simulink model "AC_DCj_iaocuo_full_TCM_THD_optimized_"  (R2024b)
settings: Solver=FixedStepDiscrete  StartTime=0.0  StopTime=0.2  FixedStep=1e-7  RelTol=1e-3
libraries: spsMosfetLib x6, spsSeriesRLCBranchLib x6, spsCurrentMeasurementLib x4, spsVoltageMeasurementLib x2, spsACVoltageSourceLib x1, slpidlib x1, dspstat3 x1, sps_lib x1, simulink x1
settings Model: Creator=YuJian  LastModifiedBy=YuJian
settings DataIOCC: ReturnWorkspaceOutputs=off

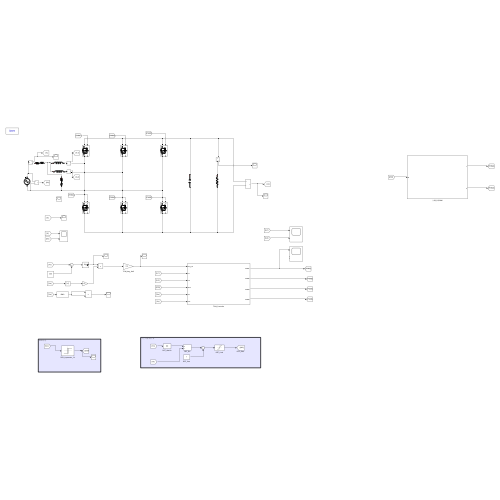
[thumbnail: Simulink's stored preview of the top-level diagram]
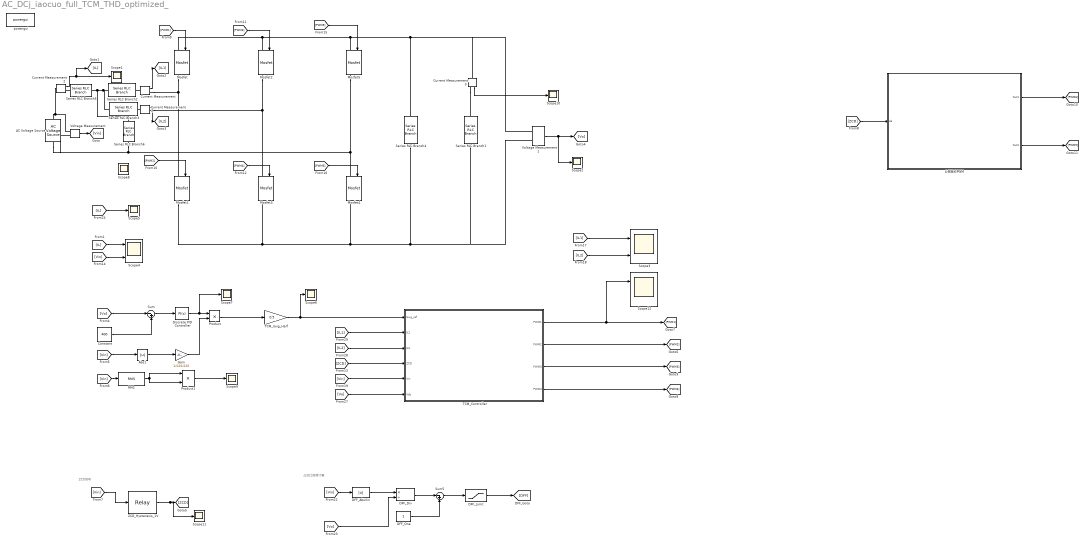
== system AC_DCj_iaocuo_full_TCM_THD_optimized_ ==
  note: 占空比前馈计算
  note: ZCD信号
  AC Voltage Source : spsACVoltageSourceLib/AC Voltage Source  Amplitude=311  Phase=0  Frequency=50  SampleTime=0  Measurements=None  BusType=swing  Pref=10e3  Qref=0  Qmin=-inf  Qmax=+inf
  Abs1 : Abs  SaturateOnIntegerOverflow=off
  Constant : Constant  Value=400
  Current Measurement{,1..3} (4 alike) : spsCurrentMeasurementLib/Current Measurement  PhasorSimulation=off  OutputType=Complex  PSBequivalent=0
  DFF_AbsVin : Abs  SaturateOnIntegerOverflow=off
  DFF_Div : Product  Inputs=*/
  DFF_Limit : Saturate  UpperLimit=1  LowerLimit=0
  DFF_One : Constant
  Discrete PID Controller : slpidlib/PID Controller  Controller=PI  Form=Parallel  TimeDomain=Discrete-time  UseExternalTs=off  SampleTime=-1  IntegratorMethod=Forward Euler  FilterMethod=Forward Euler  ControllerParametersSource=internal  P=4  I=230  UseKiTs=off  D=0  UseExternalDerivativeSource=off  N=100  UseFilter=on  TunerSelectOption=Transfer Function Based (PID Tuner App)  InitialConditionSource=internal  InitialConditionForIntegrator=5500  InitialConditionForFilter=0  DifferentiatorICPrevScaledInput=0  ExternalReset=none  TrackingMode=off  Kt=1  LimitOutput=on  SatLimitsSource=internal  UpperSaturationLimit=6500  LowerSaturationLimit=0  LinearizeAsGain=off  AntiWindupMode=clamping  Kb=1  LimitIntegrator=off  UpperIntegratorSaturationLimit=inf  LowerIntegratorSaturationLimit=-inf  POutMin=[]  POutMax=[]  IOutMin=[]  IOutMax=[]  DOutMin=[]  DOutMax=[]  NOutMin=[]  NOutMax=[]  SumOutMin=[]  SumOutMax=[]  SaturationOutMin=[]  SaturationOutMax=[]  PParamMin=[]  PParamMax=[]  IParamMin=[]  IParamMax=[]  DParamMin=[]  DParamMax=[]  NParamMin=[]  NParamMax=[]  KbParamMin=[]  KbParamMax=[]  KtParamMin=[]  KtParamMax=[]  KbOutMin=[]  KbOutMax=[]  KtOutMin=[]  KtOutMax=[]  IntegratorOutMin=[]  IntegratorOutMax=[]  FilterOutMin=[]  FilterOutMax=[]  SumI1OutMin=[]  SumI1OutMax=[]  SumI2OutMin=[]  SumI2OutMax=[]  SumI3OutMin=[]  SumI3OutMax=[]  SumI4OutMin=[]  SumI4OutMax=[]  SumDOutMin=[]  SumDOutMax=[]  DifferentiatorOutMin=[]  DifferentiatorOutMax=[]  FilterDiffOutCoefMin=[]  FilterDiffOutCoefMax=[]  ReciprocalOutMin=[]  ReciprocalOutMax=[]  SumDenOutMin=[]  SumDenOutMax=[]  SumNumOutMin=[]  SumNumOutMax=[]  DivideOutMin=[]  DivideOutMax=[]  UdiffTsProdOutMin=[]  UdiffTsProdOutMax=[]  NTsProdOutMin=[]  NTsProdOutMax=[]  UintegralTsProdOutMin=[]  UintegralTsProdOutMax=[]  UngainTsProdOutMin=[]  UngainTsProdOutMax=[]  ClampingZeroOutDataTypeStr=Inherit: Inherit via back propagation  ClampingZeroOutMin=[]  ClampingZeroOutMax=[]  FilterDenConstantOutDataTypeStr=Inherit: Inherit via back propagation  FilterDenConstantOutMin=[]  FilterDenConstantOutMax=[]  PCopyOutDataTypeStr=Inherit: Inherit via back propagation  PCopyOutMin=[]  PCopyOutMax=[]  NCopyOutDataTypeStr=Inherit: Inherit via back propagation  NCopyOutMin=[]  NCopyOutMax=[]  IntegratorContinuousStateAttributes=''  IntegratorStateMustResolveToSignalObject=off  IntegratorRTWStateStorageClass=Auto  FilterContinuousStateAttributes=''  FilterStateMustResolveToSignalObject=off  FilterRTWStateStorageClass=Auto  ParallelPVariant=InternalParameters  IdealPVariant=Disabled  IVariant=InternalParameters  DVariant=Disabled  IntegratorVariant=Discrete  SatVariant=Enabled  AWVariant=DiscClampingParallel  PCopyVariant=Disabled  TRVariant=Disabled  FdbkBlocksVariant=Forward  IdealPFdbkVariant=Disabled  SatFdbkVariant=Disabled  DerivativeFilterVariant=Disabled  NVariant=Disabled  NCopyVariant=Disabled_SignalSpec  FilterICVariant=Disabled  IntegratorICVariant=InternalICs  ExternalResetVariant=Disabled  TRSumVariant=Passthrough  SumFdbkVariant=Disabled  SumVariant=Sum_PI  TsampFilterVariant=InternalTs  TsampNgainVariant=Passthrough  TsampIntegralVariant=Disabled_SignalSpec  ExternalSaturationOutDataTypeStr=Inherit: Same as second input  DerivativeSourceVariant=Disabled  PreIntVariant=InternalPreInt
      settings: LibrarySourceBlock=simulink/Discrete/Discrete PID Controller
  Gain : Gain  Gain=1/220/220
  Mosfet{,1..5} (6 alike) : spsMosfetLib/Mosfet  Ron=0.1  Lon=0  Rd=0.01  Vfd=0  IC=0  Rs=1e5  Cs=inf  Measurements=on
  Product : Product
  Product1 : Product
  RMS : dspstat3/RMS  run=off  directionMode=Each column  dimension=1  InputProcessing=Columns as channels (frame based)  reset_popup=None
  Scope{1..2,5..11} (9 alike) : Scope
  Scope12 : Scope  NumInputPorts=2
  Scope3 : Scope  NumInputPorts=2
  Scope4 : Scope  NumInputPorts=2
  Series RLC Branch1 : spsSeriesRLCBranchLib/Series RLC Branch  LConnTagsString=__new0  RConnTagsString=__new0  BranchType=R  Resistance=29.0909  Inductance=1e-3  SetiL0=off  InitialCurrent=0  Capacitance=1e-6  Setx0=off  InitialVoltage=0  Measurements=None
  Series RLC Branch2 : spsSeriesRLCBranchLib/Series RLC Branch  LConnTagsString=__new0  RConnTagsString=__new0  BranchType=L  Resistance=1  Inductance=50e-6  SetiL0=off  InitialCurrent=0  Capacitance=1e-6  Setx0=off  InitialVoltage=0  Measurements=None
  Series RLC Branch3 : spsSeriesRLCBranchLib/Series RLC Branch  LConnTagsString=__new0  RConnTagsString=__new0  BranchType=L  Resistance=1  Inductance=50e-6  SetiL0=off  InitialCurrent=0  Capacitance=1e-6  Setx0=off  InitialVoltage=0  Measurements=None
  Series RLC Branch4 : spsSeriesRLCBranchLib/Series RLC Branch  LConnTagsString=__new0  RConnTagsString=__new0  BranchType=C  Resistance=1  Inductance=1e-3  SetiL0=off  InitialCurrent=0  Capacitance=2680e-6  Setx0=on  InitialVoltage=400  Measurements=None
  Series RLC Branch5 : spsSeriesRLCBranchLib/Series RLC Branch  LConnTagsString=__new0  RConnTagsString=__new0  BranchType=RL  Resistance=0.05  Inductance=30e-6  SetiL0=off  InitialCurrent=0  Capacitance=1e-6  Setx0=off  InitialVoltage=0  Measurements=None
  Series RLC Branch6 : spsSeriesRLCBranchLib/Series RLC Branch  LConnTagsString=__new0  RConnTagsString=__new0  BranchType=RC  Resistance=1  Inductance=30e-6  SetiL0=off  InitialCurrent=0  Capacitance=2.2e-6  Setx0=off  InitialVoltage=0  Measurements=None
  Sum : Sum  Inputs=|-+
  Sum5 : Sum  Inputs=|-+
  TCM_Controller : Subsystem
  TCM_Iavg_Half : Gain  Gain=0.5
  Voltage Measurement : spsVoltageMeasurementLib/Voltage Measurement  PhasorSimulation=off  OutputType=Complex  PSBequivalent=0
  Voltage Measurement1 : spsVoltageMeasurementLib/Voltage Measurement  PhasorSimulation=off  OutputType=Complex  PSBequivalent=0
  ZCD_Hysteresis_1V : Relay  OnSwitchValue=1  OffSwitchValue=-1  OutDataTypeStr=boolean
  powergui : sps_lib/powergui  Priority=1  SimulationMode=Discrete  SampleTime=1e-7  frequency=60  Iterations=50  frequencyindice=50  Pbase=100e6  ErrMax=1e-4  UnitsV=kV  UnitsW=MW  buscounter=0  FunctionMessages=off  echomessages=off  EnableUseOfTLC=off  CurrentSourceSwitches=off  DisableSnubberDevices=off  DisableRonSwitches=off  DisableVfSwitches=off  DisplayEquations=off  AutomaticDiscreteSolvers=off  SolverType=Tustin/Backward Euler (TBE)  Interpol=off  ExternalGateDelay=off  methode=off  Ts=100  x0status=blocks  SPID=on  SwTol=0  HookPort=off  NonlinearTolerance=1e-4  nMaxIteration=100  ContinueOnMaxIteration=off  RestoreLinks=warning  ResistiveCurrentMeasurement=off  Frange=[0:2:500]  Ylog=off  Xlog=on  ShowGrid=off  save=off  variable=ZData  structure=0  ZoomFFT=off  StartTime=0.0  cycles=1  DisplayStyle=1  fundamental=60  FreqAxis=off  MaxFrequency=1000  frequencyindicesteady=1  RmsSteady=1  display=off
  公频驱动PWM : Subsystem
  wires:
  Current Measurement2/1 -> Scope1/1, [IL]
  Current Measurement/1 -> [IL1]
  Current Measurement1/1 -> [IL2]
  Voltage Measurement1/1 -> Scope2/1, [Vo]
  Voltage Measurement/1 -> [Vin]
  Constant/1 -> Sum/2
  [Vo] -> Sum/1
  Sum/1 -> Discrete PID Controller/1
  Discrete PID Controller/1 -> Scope7/1, Product/1
  Gain/1 -> Product/2
  [Vin] -> RMS/1
  [PWM4] -> Mosfet3/1
  [PWM3] -> Mosfet2/1
  [PWM2] -> Mosfet1/1
  [PWM1] -> Mosfet/1
  [PWM5] -> Mosfet5/1
  [PWM6] -> Mosfet4/1
  [IL1] -> Scope3/1
  [IL2] -> Scope3/2
  Product1/1 -> Scope9/1
  Current Measurement3/1 -> Scope10/1
  [Vin] -> Abs1/1
  Abs1/1 -> Gain/1
  DFF_AbsVin/1 -> DFF_Div/1
  Sum5/1 -> DFF_Limit/1
  DFF_Limit/1 -> [DFF]
  [Vin] -> DFF_AbsVin/1
  [Vo] -> DFF_Div/2
  公频驱动PWM/1(Out1) -> [PWM6]
  公频驱动PWM/2(Out2) -> [PWM5]
  [ZCD] -> 公频驱动PWM/1(da)
  [ZCD] -> TCM_Controller/4(ZCD)
  DFF_One/1 -> Sum5/2
  DFF_Div/1 -> Sum5/1
  [IL] -> Scope4/1
  [Vin] -> Scope4/2
  Product/1 -> TCM_Iavg_Half/1
  RMS/1 -> Product1/2, Product1/1
  [IL] -> Scope5/1
  [Vin] -> ZCD_Hysteresis_1V/1
  ZCD_Hysteresis_1V/1 -> [ZCD], Scope11/1
  TCM_Controller/1(PWM1) -> Scope12/1, [PWM1]
  TCM_Controller/2(PWM2) -> [PWM2]
  TCM_Controller/3(PWM3) -> [PWM3]
  TCM_Controller/4(PWM4) -> [PWM4]
  TCM_Iavg_Half/1 -> Scope6/1, TCM_Controller/1(Iavg_ref)
  [Vin] -> TCM_Controller/5(Vin)
  [Vo] -> TCM_Controller/6(Vdc)
  [IL2] -> TCM_Controller/3(IL2)
  [IL1] -> TCM_Controller/2(IL1)
  connections:
  Mosfet/RConn1 -- Current Measurement/RConn1 -- Mosfet1/LConn1
  Mosfet5/RConn1 -- Series RLC Branch6/RConn1 -- Voltage Measurement/LConn2 -- AC Voltage Source/LConn1 -- Mosfet4/LConn1
  Mosfet/LConn1 -- Mosfet2/LConn1 -- Current Measurement3/LConn1 -- Voltage Measurement1/LConn1 -- Series RLC Branch4/LConn1 -- Mosfet5/LConn1
  Mosfet1/RConn1 -- Voltage Measurement1/LConn2 -- Series RLC Branch1/RConn1 -- Series RLC Branch4/RConn1 -- Mosfet4/RConn1 -- Mosfet3/RConn1
  AC Voltage Source/RConn1 -- Voltage Measurement/LConn1 -- Current Measurement2/LConn1
  Mosfet2/RConn1 -- Current Measurement1/RConn1 -- Mosfet3/LConn1
  Current Measurement/LConn1 -- Series RLC Branch2/RConn1
  Series RLC Branch3/RConn1 -- Current Measurement1/LConn1
  Current Measurement3/RConn1 -- Series RLC Branch1/LConn1
  Series RLC Branch5/LConn1 -- Current Measurement2/RConn1
  Series RLC Branch5/RConn1 -- Series RLC Branch3/LConn1 -- Series RLC Branch2/LConn1 -- Series RLC Branch6/LConn1

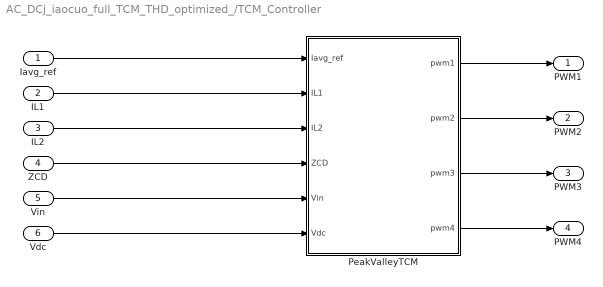
== system AC_DCj_iaocuo_full_TCM_THD_optimized_/TCM_Controller ==
  Iavg_ref : Inport
  IL1 : Inport  Port=2
  IL2 : Inport  Port=3
  ZCD : Inport  Port=4
  Vin : Inport  Port=5
  Vdc : Inport  Port=6
  PeakValleyTCM : MATLAB Function  TreatAsAtomicUnit=on
  PWM1 : Outport
  PWM2 : Outport  Port=2
  PWM3 : Outport  Port=3
  PWM4 : Outport  Port=4
  wires:
  Iavg_ref/1 -> PeakValleyTCM/1(Iavg_ref)
  IL1/1 -> PeakValleyTCM/2(IL1)
  IL2/1 -> PeakValleyTCM/3(IL2)
  ZCD/1 -> PeakValleyTCM/4(ZCD)
  Vin/1 -> PeakValleyTCM/5(Vin)
  PeakValleyTCM/1(pwm1) -> PWM1/1
  PeakValleyTCM/2(pwm2) -> PWM2/1
  PeakValleyTCM/3(pwm3) -> PWM3/1
  PeakValleyTCM/4(pwm4) -> PWM4/1
  Vdc/1 -> PeakValleyTCM/6(Vdc)

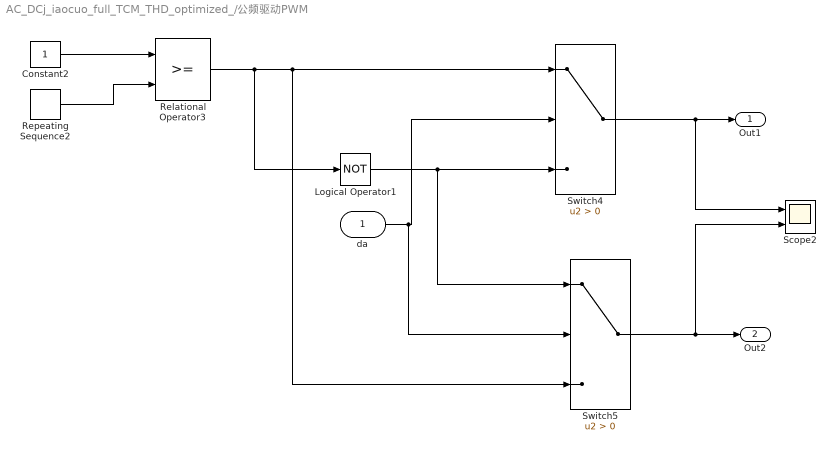
== system AC_DCj_iaocuo_full_TCM_THD_optimized_/公频驱动PWM ==
  da : Inport
  Constant2 : Constant
  Logical Operator1 : Logic  Operator=NOT  AllPortsSameDT=off  OutDataTypeStr=boolean
  Relational Operator3 : RelationalOperator  OutDataTypeStr=boolean  RndMeth=Simplest  InputSameDT=off
  Repeating Sequence2 : simulink/Sources/Repeating Sequence  rep_seq_t=[0 0.00001 0.00002]  rep_seq_y=[0 1 0]
  Scope2 : Scope  NumInputPorts=2
  Switch4 : Switch  Criteria=u2 > Threshold  SaturateOnIntegerOverflow=off  InputSameDT=off
  Switch5 : Switch  Criteria=u2 > Threshold  SaturateOnIntegerOverflow=off  InputSameDT=off
  Out1 : Outport
  Out2 : Outport  Port=2
  wires:
  Repeating Sequence2/1 -> Relational Operator3/2
  da/1 -> Switch5/2, Switch4/2
  Relational Operator3/1 -> Logical Operator1/1, Switch5/3, Switch4/1
  Switch4/1 -> Scope2/1, Out1/1
  Switch5/1 -> Scope2/2, Out2/1
  Logical Operator1/1 -> Switch5/1, Switch4/3
  Constant2/1 -> Relational Operator3/1

== matlab function AC_DCj_iaocuo_full_TCM_THD_optimized_/TCM_Controller/PeakValleyTCM ==
  data: Iavg_ref input; pwm1 output; IL1 input; IL2 input; ZCD input; Vin input; pwm2 output; pwm3 output; pwm4 output; Vdc input
function [pwm1,pwm2,pwm3,pwm4] = fcn(Iavg_ref,IL1,IL2,ZCD,Vin,Vdc)
% 完整两相交错 TCM 高频控制器（实际相位闭环版本）。
%
% 控制原则：
% 1. 两相都根据自己的电感电流独立进行峰值/谷值换相；
% 2. 两相每次换相只保留固定死区，不在负谷值后增加长时间全关断；
% 3. 第一相作为周期基准，第二相实际周期起点与目标 180 度位置比较；
% 4. 相位误差只对第二相峰值作小幅、受限的逐周期修正；
% 5. 启动和工频换向后，第二相先延迟预测的半个周期再起振。
%
% 输入说明：
% Iavg_ref：每相平均电流给定，不是两相总电流给定。
% IL1、IL2：两相电感实际电流。
% ZCD：保留接口；当前仿真直接用 IL1、IL2 完成峰谷检测。
% Vin：输入电压，用于半周判断、过零保护和启动周期预测。
% Vdc：母线电压，用于升压有效性保护和 ZVS 谷值调节。
%
% 正半周：PWM2/PWM4 控制上升段，PWM1/PWM3 控制下降段。
% 负半周：PWM1/PWM3 控制上升段，PWM2/PWM4 控制下降段。

persistent rise1 rise2 dead1 dead2 age1 age2
persistent polarityOld controlWasDisabled sampleCounter
persistent lastCycle1 period1Filt halfPeriod
persistent lastCycle2 period2Filt
persistent phase2Started startupDelay2 phaseErrFilt
persistent cycleSum1 cycleSum2 cycleCount1 cycleCount2
persistent avgMeasured1 avgMeasured2 trimIntCommon

% -------------------- 固定参数 --------------------
Ts = 1e-7;                    % 控制器执行周期：0.1 us
Lphase = 50e-6;               % 每相升压电感：50 uH，仅用于启动周期预测
IzvsMax = 0.10;               % 最大 ZVS 负谷值电流；以降低高频纹波为优先
% 注意：当前功率级 MOS 模型未完整建立 Coss/寄生参数，0.10 A 是仿真纹波优化值；硬件需按 Vds 波形重新核定 ZVS 负谷值。
Vzero = 1.0;                  % 过零屏蔽阈值
Vfull = 25.0;                 % 输入电压达到该值后使用完整 Izvs
Vmargin = 10.0;               % Vdc 必须高于 |Vin| 的裕量
IavgMax = 22.0;               % 单相平均电流给定限幅
minStateSamples = uint32(1);  % 峰谷检测最短保持：0.1 us
maxStateSamples = uint32(250);% 单个上升/下降段最大时间：25 us
baseDeadSamples = uint32(1);  % 每次高频换相固定全关断死区：0.1 us
minPeriodSamples = 20.0;      % 有效主相周期下限：2 us
maxPeriodSamples = 320.0;     % 有效主相周期上限：32 us
periodFilter = 0.25;          % 主相周期低通更新系数
phaseFilter = 0.30;           % 相位误差低通更新系数
Kphase = 0.040;               % 相位误差到第二相峰值修正：A/采样点
phaseTrimMax = 1.50;          % 第二相相位修正最大幅度
Kperiod = 0.015;              % 第二相周期误差到峰值修正：A/采样点
periodTrimMax = 0.60;         % 周期匹配修正限幅
startupPhaseBias = 6.0;       % 低 Izvs 时的启动相位补偿：0.6 us
KavgP = 0.65;                 % 周期平均电流修正比例系数
KavgI = 0.08;                 % 周期平均电流修正积分系数
trimMax = 3.0;                % 平均电流峰值修正最大幅度
Kbalance = 0.20;              % 两相周期平均电流的小幅比例均流
balanceTrimMax = 0.60;        % 均流修正限幅，避免干扰相位环

% -------------------- 初始化 --------------------
if isempty(rise1)
    rise1 = true; rise2 = true;
    dead1 = baseDeadSamples; dead2 = baseDeadSamples;
    age1 = uint32(0); age2 = uint32(0);
    polarityOld = (Vin >= 0);
    controlWasDisabled = true;
    sampleCounter = 0.0;
    lastCycle1 = 0.0;
    lastCycle2 = 0.0;
    period1Filt = 110.0;      % 约 11 us，接近当前功率级的典型周期
    period2Filt = period1Filt;
    halfPeriod = 0.5*period1Filt;
    phase2Started = false;
    startupDelay2 = uint32(max(0,round(halfPeriod+startupPhaseBias)));
    phaseErrFilt = 0.0;
    cycleSum1 = 0.0; cycleSum2 = 0.0;
    cycleCount1 = uint32(0); cycleCount2 = uint32(0);
    avgMeasured1 = min(max(abs(Iavg_ref),0.0),IavgMax);
    avgMeasured2 = avgMeasured1;
    trimIntCommon = 0.0;
end
sampleCounter = sampleCounter + 1.0;

% 默认安全状态：只有状态机明确允许时才输出门极。
pwm1 = 0.0; pwm2 = 0.0; pwm3 = 0.0; pwm4 = 0.0;

% -------------------- 电流峰值和 ZVS 谷值 --------------------
Iavg = min(max(abs(Iavg_ref),0.0),IavgMax);
lineFactor = (abs(Vin)-Vzero)/(Vfull-Vzero);
lineFactor = min(max(lineFactor,0.0),1.0);
vdcFactor = min(max(Vdc/400.0,0.70),1.30);
Izvs = IzvsMax*lineFactor*vdcFactor;
IpkBase = 2.0*Iavg + Izvs;

% -------------------- 过零及升压有效性保护 --------------------
polarity = (Vin >= 0);
disableControl = (abs(Vin) < Vzero) || (Vdc <= abs(Vin)+Vmargin);
if polarity ~= polarityOld
    disableControl = true;
end

if disableControl
    % 过零或升压条件不满足时，四个高频管全部关闭并复位半周状态。
    rise1 = true; rise2 = true;
    dead1 = baseDeadSamples; dead2 = baseDeadSamples;
    age1 = uint32(0); age2 = uint32(0);
    polarityOld = polarity;
    controlWasDisabled = true;
    lastCycle1 = 0.0;
    lastCycle2 = 0.0;
    period2Filt = period1Filt;
    phase2Started = false;
    phaseErrFilt = 0.0;
    cycleSum1 = 0.0; cycleSum2 = 0.0;
    cycleCount1 = uint32(0); cycleCount2 = uint32(0);
    avgMeasured1 = Iavg; avgMeasured2 = Iavg;
    trimIntCommon = 0.0;
else
    % 每个工频半周重新启动时，根据当前 Vin、Vdc 和电流给定预测 TCM 周期。
    % 第二相只在这里等待半周期；此时电流接近零，不会在负谷值后继续变负。
    if controlWasDisabled
        deltaI = IpkBase + Izvs;
        riseSamples = Lphase*deltaI/(max(abs(Vin),Vzero)*Ts);
        fallSamples = Lphase*deltaI/(max(Vdc-abs(Vin),Vmargin)*Ts);
        predictedPeriod = riseSamples + fallSamples + 2.0*double(baseDeadSamples);
        predictedPeriod = min(max(predictedPeriod,minPeriodSamples),maxPeriodSamples);
        period1Filt = predictedPeriod;
        halfPeriod = 0.5*period1Filt;
        startupDelay2 = uint32(max(0,round(halfPeriod+startupPhaseBias)));
        phase2Started = false;
        lastCycle1 = 0.0;
        lastCycle2 = 0.0;
        period2Filt = period1Filt;
        phaseErrFilt = 0.0;
        controlWasDisabled = false;
    end

    % 将负半周电流折算到统一的正方向。
    x1 = IL1; x2 = IL2;
    if ~polarity
        x1 = -IL1; x2 = -IL2;
    end

    % -------------------- 公共平均电流修正 --------------------
    % 两相使用同一个幅值 PI，保持总电流跟踪 Iavg_ref。
    % 不再给第二相使用独立积分器：独立积分器会把相位环
    % 对 Ipk2 的修正抵消，导致实际交错长期停在约 160 度。
    trimLimit = min(trimMax,0.25+0.25*Iavg);
    avgMeasuredCommon = 0.5*(avgMeasured1+avgMeasured2);
    errCommon = Iavg-avgMeasuredCommon;
    peakTrimCommon = min(max(KavgP*errCommon+trimIntCommon, ...
        -trimLimit),trimLimit);

    % 均流只用小幅比例修正，不使用积分，因此不会“顶住”相位环。
    balanceTrim = Kbalance*(avgMeasured1-avgMeasured2);
    balanceTrim = min(max(balanceTrim,-balanceTrimMax),balanceTrimMax);

    % 相位闭环只做小幅修正，避免为了锁相破坏电流幅值。
    phaseLimit = min(phaseTrimMax,0.15+0.12*Iavg);
    phasePeakTrim = min(max(-Kphase*phaseErrFilt,-phaseLimit),phaseLimit);
    % 周期匹配：如果第二相周期偏长，减小其峰值；偏短则增大峰值。
    % 这一项直接抑制周期漂移，比只根据相位误差调节更稳定。
    periodError = period2Filt-period1Filt;
    periodPeakTrim = min(max(-Kperiod*periodError, ...
        -periodTrimMax),periodTrimMax);
    Ipk1 = max(Izvs+0.05,IpkBase+peakTrimCommon);
    Ipk2 = max(Izvs+0.05,IpkBase+peakTrimCommon+balanceTrim+ ...
        phasePeakTrim+periodPeakTrim);

    % -------------------- 第一相：周期基准相 --------------------
    cycleSum1 = cycleSum1+x1;
    cycleCount1 = cycleCount1+uint32(1);
    [rise1,dead1,age1,cycleStart1] = update_state( ...
        rise1,dead1,age1,x1,Ipk1,Izvs,minStateSamples, ...
        maxStateSamples,baseDeadSamples);

    if cycleStart1
        if cycleCount1 > 0
            avgMeasured1 = cycleSum1/double(cycleCount1);
            trimIntCommon = min(max(trimIntCommon+KavgI*(Iavg- ...
                0.5*(avgMeasured1+avgMeasured2)), ...
                -trimLimit),trimLimit);
        end
        cycleSum1 = 0.0; cycleCount1 = uint32(0);

        % 相邻两个第一相周期起点之间的时间就是实际主相周期。
        if lastCycle1 > 0.0
            measuredPeriod = sampleCounter-lastCycle1;
            if measuredPeriod >= minPeriodSamples && measuredPeriod <= maxPeriodSamples
                period1Filt = (1.0-periodFilter)*period1Filt + ...
                    periodFilter*measuredPeriod;
                halfPeriod = 0.5*period1Filt;
            end
        end
        lastCycle1 = sampleCounter;
    end

    % -------------------- 第二相启动 --------------------
    % 只在半周启动时延迟一次，使第二相初始位置接近 180 度。
    if ~phase2Started
        rise2 = true;
        dead2 = baseDeadSamples;
        age2 = uint32(0);
        cycleSum2 = 0.0; cycleCount2 = uint32(0);
        avgMeasured2 = Iavg;
        if startupDelay2 > 0
            startupDelay2 = startupDelay2-uint32(1);
        else
            phase2Started = true;
        end
    else
        % -------------------- 第二相：独立峰谷控制 --------------------
        cycleSum2 = cycleSum2+x2;
        cycleCount2 = cycleCount2+uint32(1);
        [rise2,dead2,age2,cycleStart2] = update_state( ...
            rise2,dead2,age2,x2,Ipk2,Izvs,minStateSamples, ...
            maxStateSamples,baseDeadSamples);

        if cycleStart2
            if cycleCount2 > 0
                avgMeasured2 = cycleSum2/double(cycleCount2);
            end
            cycleSum2 = 0.0; cycleCount2 = uint32(0);

            % 测量第二相两个周期起点的间隔，用于周期匹配。
            if lastCycle2 > 0.0
                measuredPeriod2 = sampleCounter-lastCycle2;
                if measuredPeriod2 >= minPeriodSamples && ...
                        measuredPeriod2 <= maxPeriodSamples
                    period2Filt = (1.0-periodFilter)*period2Filt + ...
                        periodFilter*measuredPeriod2;
                end
            end
            lastCycle2 = sampleCounter;

            % 捕获第二相相对于最近第一相周期起点的实际位置。
            % 目标位置为 period1Filt/2，即 180 度。
            if lastCycle1 > 0.0
                phasePosition = sampleCounter-lastCycle1;
                if phasePosition >= period1Filt
                    phasePosition = phasePosition- ...
                        floor(phasePosition/period1Filt)*period1Filt;
                end
                phaseError = phasePosition-halfPeriod;
                phaseErrFilt = (1.0-phaseFilter)*phaseErrFilt + ...
                    phaseFilter*phaseError;
            end
        end
    end

    % -------------------- 门极译码 --------------------
    if dead1 == 0
        if polarity
            pwm2 = double(rise1);      % 正半周第一相上升管
            pwm1 = double(~rise1);     % 正半周第一相下降管
        else
            pwm1 = double(rise1);      % 负半周第一相上升管
            pwm2 = double(~rise1);     % 负半周第一相下降管
        end
    end

    if phase2Started && dead2 == 0
        if polarity
            pwm4 = double(rise2);      % 正半周第二相上升管
            pwm3 = double(~rise2);     % 正半周第二相下降管
        else
            pwm3 = double(rise2);      % 负半周第二相上升管
            pwm4 = double(~rise2);     % 负半周第二相下降管
        end
    end
end
end

function [rise,dead,age,cycleStart] = update_state( ...
    rise,dead,age,x,Ipk,Izvs,minAge,maxAge,deadSamples)
% 单相 TCM 峰谷状态机。
% rise=true ：上升段达到 Ipk 后切换到下降段。
% rise=false：下降段达到 -Izvs 后切换到下一上升段。
% 两个换相方向都只加入 deadSamples 固定死区。
cycleStart = false;

if dead > 0
    dead = dead-uint32(1);
    age = uint32(0);
    return
end

age = age+uint32(1);
if age < minAge
    return
end

forceSwitch = (age >= maxAge);
if rise
    if forceSwitch || x >= Ipk
        rise = false;
        dead = deadSamples;
        age = uint32(0);
    end
else
    if forceSwitch || x <= -Izvs
        rise = true;
        dead = deadSamples;
        age = uint32(0);
        cycleStart = true;
    end
end
end
